simulink model "mavsim_trim"  (R2025a)
settings: Solver=ode45  StartTime=0.0  StopTime=10000  RelTol=1e-3  EnableMultiTasking=on
values from neighbouring files (symbols this model uses):
  P = evalin('base', 'P')    [diagnostico_energia.m]    (also in graficas_video.m)
undefined symbols (not defined in the file or in its folder): fym
settings Model: Creator=beard  LastModifiedBy=anton
settings SolverCC: AlgebraicLoopSolver=TrustRegion
settings DataIOCC: LimitDataPoints=on  SaveFormat=Array  SignalLoggingSaveFormat=ModelDataLogs  ReturnWorkspaceOutputs=off
settings OptimizationCC: ExpressionDepthLimit=2147483647.0  InitFltsAndDblsToZero=on  LifeSpan=inf
settings DebuggingCC: UnderspecifiedInitializationDetection=Classic  MergeDetectMultiDrivingBlocksExec=none  SolverPrmCheckMsg=warning  FcnCallInpInsideContextMsg=warning  UnconnectedInputMsg=warning  UnconnectedOutputMsg=warning  UnconnectedLineMsg=warning  StateNameClashWarn=warning  SFUnexpectedBacktrackingDiag=warning  SFNoUnconditionalDefaultTransitionDiag=warning  ArithmeticOperatorsInVariantConditions=warning
settings HardwareCC: ProdBitPerPointer=32.0  ProdBitPerSizeT=32.0  ProdBitPerPtrDiffT=32.0  ProdLargestAtomicFloat=None  ProdIntDivRoundTo=Undefined  ProdEndianess=Unspecified  ProdWordSize=32.0  ProdHWDeviceType=32-bit Generic
settings ModelReferenceCC: EnableRefExpFcnMdlSchedulingChecks=on  PropagateSignalLabelsOutOfModel=off
settings SFSimCC: SimUseLocalCustomCode=off  CustomCodeUndefinedFunction=UseInterfaceOnly
settings RTWCC: RTWUseLocalCustomCode=off  GPUComputeCapability=3.5  DLArmComputeVersion=19.05
settings CodeAppCC: StateflowObjectComments=on
settings GRTTargetCC: TargetLangStandard=C89/C90 (ANSI)  CombineOutputUpdateFcns=off  GRTInterface=on
settings ConfigComp: CovMetricSettings=dw  CovSaveCumulativeToWorkspaceVar=on  CovSaveSingleToWorkspaceVar=on  CovExternalEMLEnable=off  CovSFcnEnable=off

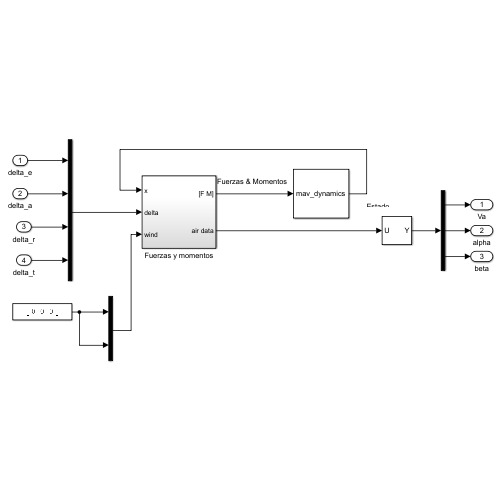
[thumbnail: Simulink's stored preview of the top-level diagram]
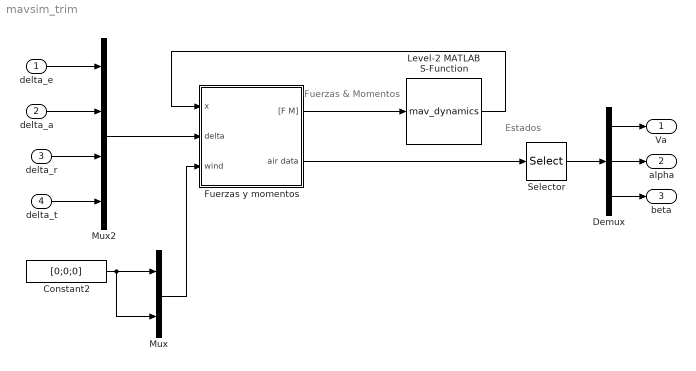
== system mavsim_trim ==
  note: Fuerzas & Momentos
  note: Estados
  delta_e : Inport
  delta_a : Inport  Port=2
  delta_r : Inport  Port=3
  delta_t : Inport  Port=4
  Constant2 : Constant  Value=[0;0;0]
  Demux : Demux  Outputs=3
  Fuerzas y momentos : Subsystem
  Level-2 MATLAB S-Function : M-S-Function  FunctionName=mav_dynamics  Parameters=mass,Jx,Jy,Jz,Jxz,pn0,pe0,pd0,u0,v0,w0,phi0,theta0,psi0,p0,q0,r0  mask{mass=P.mass, Jx=P.Jx, Jy=P.Jy, Jz=P.Jz, Jxz=P.Jxz, pn0=P.pn0, pe0=P.pe0, pd0=P.pd0, u0=P.u0, v0=P.v0, w0=P.w0, phi0=P.phi0, theta0=P.theta0, psi0=P.psi0, p0=P.p0, q0=P.q0, r0=P.r0}
  Mux : Mux  Inputs=2
  Mux2 : Mux
  Selector : Selector  InputPortWidth=6  IndexOptions=Index vector (dialog)  Indices=[1 2 3]  OutputSizes=1
  Va : Outport
  alpha : Outport  Port=2
  beta : Outport  Port=3
  wires:
  Constant2/1 -> Mux/1, Mux/2
  delta_e/1 -> Mux2/1
  delta_a/1 -> Mux2/2
  delta_r/1 -> Mux2/3
  delta_t/1 -> Mux2/4
  Level-2 MATLAB S-Function/1 -> Fuerzas y momentos/1(x)
  Mux2/1 -> Fuerzas y momentos/2(delta)
  Fuerzas y momentos/1("[F M]") -> Level-2 MATLAB S-Function/1
  Mux/1 -> Fuerzas y momentos/3(wind)
  Fuerzas y momentos/2(air data) -> Selector/1
  Selector/1 -> Demux/1
  Demux/1 -> Va/1
  Demux/2 -> alpha/1
  Demux/3 -> beta/1

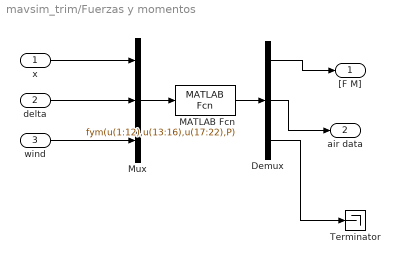
== system mavsim_trim/Fuerzas y momentos ==
  x : Inport
  delta : Inport  Port=2
  wind : Inport  Port=3
  Demux : Demux  Outputs=[6;6;2]
  MATLAB Fcn : MATLABFcn  MATLABFcn=fym(u(1:12),u(13:16),u(17:22),P)  OutputDimensions=14
  Mux : Mux  Inputs=3
  Terminator : Terminator
  "[F M]" : Outport
  air data : Outport  Port=2
  wires:
  Demux/2 -> air data/1
  Mux/1 -> MATLAB Fcn/1
  Demux/1 -> "[F M]"/1
  MATLAB Fcn/1 -> Demux/1
  wind/1 -> Mux/3
  delta/1 -> Mux/2
  x/1 -> Mux/1
  Demux/3 -> Terminator/1
